simulink model "DCMotor"  (R2024b)
settings: Solver=VariableStepAuto  StartTime=0.0  StopTime=0.2  RelTol=1e-3
values from neighbouring files (symbols this model uses):
  b = 0    [DC_MotorEquation_Encoder_Parameters.m]    (also in param.m = 0.000180072449898)
  Gmot = tf([Km],[L*J R*J+b*L Km*Km+b*R])    [param.m]
  GmotInv = GmotInv*pole1*pole1    [param.m]
  GmotInvz = c2d(GmotInv,TSample)    [param.m]
  J = 0.352e-4    (= 3.52e-05)    [DC_MotorEquation_Encoder_Parameters.m]    (also in param.m)
  Km = 0.11    [DC_MotorEquation_Encoder_Parameters.m]    (also in param.m)
  L = 4.1e-3    (= 0.0041)    [DC_MotorEquation_Encoder_Parameters.m]    (also in param.m)
  R = 3.2    [DC_MotorEquation_Encoder_Parameters.m]    (also in param.m)
  RadToRpm = 60/(2*pi)    (= 9.54929658551)    [BaseModelForControl_Parameters.m]    (also in DC_MotorEquation_Encoder_Parameters.m; param.m)
undefined symbols (not defined in the file or in its folder): dspblkCoreblockFVToolHelper, gcbh
settings Model: Creator=student  LastModifiedBy=student

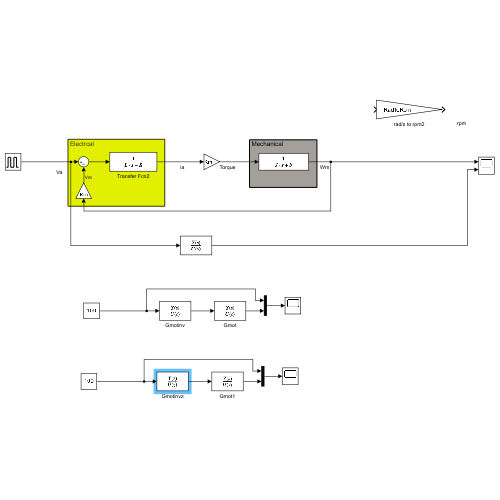
[thumbnail: Simulink's stored preview of the top-level diagram]
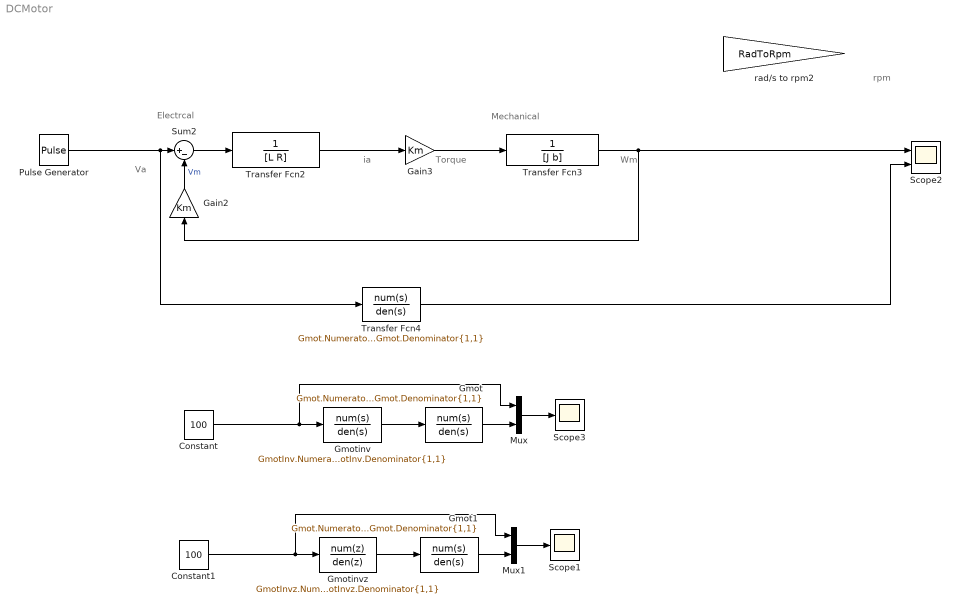
== system DCMotor ==
  note: Wm
  note: Torque
  note: Electrcal
  note: Mechanical
  note: Va
  note: ia
  note: rpm
  Constant : Constant  Value=100
  Constant1 : Constant  Value=100
  Gain2 : Gain  Gain=Km
  Gain3 : Gain  Gain=Km
  Gmot : TransferFcn  Numerator=Gmot.Numerator{1,1}  Denominator=Gmot.Denominator{1,1}
  Gmot1 : TransferFcn  Numerator=Gmot.Numerator{1,1}  Denominator=Gmot.Denominator{1,1}
  Gmotinv : TransferFcn  Numerator=GmotInv.Numerator{1,1}  Denominator=GmotInv.Denominator{1,1}
  Gmotinvz : DiscreteTransferFcn  LoadFcn=dspblkCoreblockFVToolHelper(gcbh,'load');  Numerator=GmotInvz.Numerator{1,1}  Denominator=GmotInvz.Denominator{1,1}
      settings: CopyFcn=dspblkCoreblockFVToolHelper(gcbh,'copy');  DeleteFcn=dspblkCoreblockFVToolHelper(gcbh,'close');  ModelCloseFcn=dspblkCoreblockFVToolHelper(gcbh,'close');  PreSaveFcn=dspblkCoreblockFVToolHelper(gcbh,'presave');  PostSaveFcn=dspblkCoreblockFVToolHelper(gcbh,'postsave');  CloseFcn=dspblkCoreblockFVToolHelper(gcbh,'close');
  Mux : Mux  Inputs=2
  Mux1 : Mux  Inputs=2
  Pulse Generator : DiscretePulseGenerator  PulseType=Time based  Amplitude=24  Period=0.001  PulseWidth=50
  Scope1 : Scope
  Scope2 : Scope  NumInputPorts=2
  Scope3 : Scope
  Sum2 : Sum  Inputs=|+-
  Transfer Fcn2 : TransferFcn  Denominator=[L R]
  Transfer Fcn3 : TransferFcn  Denominator=[J b]
  Transfer Fcn4 : TransferFcn  Numerator=Gmot.Numerator{1,1}  Denominator=Gmot.Denominator{1,1}
  rad/s to rpm2 : Gain  Gain=RadToRpm
  wires:
  Gain3/1 -> Transfer Fcn3/1
  Sum2/1 -> Transfer Fcn2/1
  Pulse Generator/1 -> Transfer Fcn4/1, Sum2/1
  Transfer Fcn2/1 -> Gain3/1
  Transfer Fcn3/1 -> Scope2/1, Gain2/1
  Gain2/1 -> Sum2/2  "Vm"
  Transfer Fcn4/1 -> Scope2/2
  Gmotinv/1 -> Gmot/1
  Gmot/1 -> Mux/2
  Mux/1 -> Scope3/1
  Constant/1 -> Mux/1, Gmotinv/1
  Constant1/1 -> Gmotinvz/1, Mux1/1
  Mux1/1 -> Scope1/1
  Gmot1/1 -> Mux1/2
  Gmotinvz/1 -> Gmot1/1
